simulink model "d_current_controller_discrete"  (R2025b)
settings: Solver=FixedStepDiscrete  FixedStep=control.currentLoopPeriod_s
undefined symbols (not defined in the file): control, DiscIntNeverNeededParam
settings Model: Creator=semih  LastModifiedBy=Semih
settings SFSimCC: SimGPUStackLimitPerThread=51200  SimGPUMallocThreshold=200
settings RTWCC: GPUStackLimitPerThread=51200  GPUMallocThreshold=200
settings GRTTargetCC: CombineOutputUpdateFcns=off

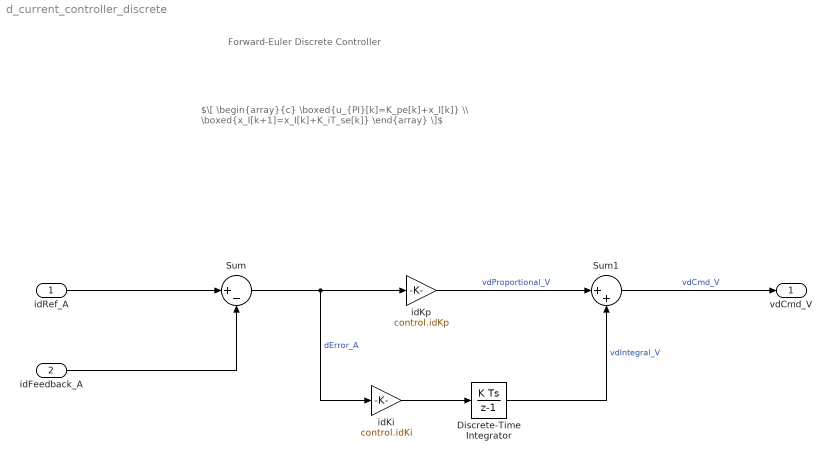
== system d_current_controller_discrete ==
  note: Forward-Euler Discrete Controller
  note: $\[ \begin{array}{c} \boxed{u_{PI}[k]=K_pe[k]+x_I[k]} \\ \boxed{x_I[k+1]=x_I[k]+K_iT_se[k]} \end{array} \]$
  idRef_A : Inport
  idFeedback_A : Inport  Port=2
  Discrete-Time Integrator : DiscreteIntegrator  SampleTime=control.currentLoopPeriod_s  ICPrevOutput=DiscIntNeverNeededParam  ICPrevScaledInput=DiscIntNeverNeededParam
  Sum : Sum  Inputs=|+-
  Sum1 : Sum  Inputs=|++
  idKi : Gain  Gain=control.idKi
  idKp : Gain  Gain=control.idKp
  vdCmd_V : Outport
  wires:
  idRef_A/1 -> Sum/1
  idFeedback_A/1 -> Sum/2
  Sum/1 -> idKp/1, idKi/1  "dError_A"
  idKi/1 -> Discrete-Time Integrator/1
  Sum1/1 -> vdCmd_V/1  "vdCmd_V"
  idKp/1 -> Sum1/1  "vdProportional_V"
  Discrete-Time Integrator/1 -> Sum1/2  "vdIntegral_V"
